simulink model "afe_inv_psm_with_hf_models"  (R2026a)
settings: Solver=ode23tb  StopTime=simlength  FixedStep=tc  MaxStep=glb_time.tc
values from neighbouring files (symbols this model uses):
  afe_ctrl = ctrl_afe_setup(glb_time.ts_afe, grid_emu.omega_grid_nom)    [init_model.m]
  afe_pwm_phase_shift_mod1 = 0    [init_model.m]
  CTRPIFF_CLIP_RELEASE = 0.001    [init_model.m]
  DThs_init = 0    [init_model.m]
  filters = setup_global_filters(glb_time.ts_afe, glb_time.ts_inv, glb_time.ts_dab, glb_time.tc)    [init_model.m]
  frt_data = frt_settings(test_index, test_subindex, asymmetric_error_type,      enable_frt_1, enable_frt_2, start_time_LVRT, deepPOSxi, deepPOSeta, deepNEGxi, deepNEGeta)    [init_model.m]
  glb_time = timing_setup(fpwm_afe, trgo_afe, fpwm_inv, trgo_inv, fpwm_single_phase_inv, trgo_single_phase_inv, fpwm_dab, trgo_dab,      fpwm_psfbc, trgo_psfbc, fpwm_isop_rail, trgo_isop_rail, fpwm_cllc, trgo_cllc, t_measure, tc_factor, tc_decimation, delay_pwm, dead_time_afe,      dead_time_inv, dead_time_single_phase_inv, dead_time_dab, dead_time_psfbc, dead_time_isop_rail, dead_time_cllc)    [init_model.m]
  grid_emu = grid_three_phase_emulator('Dyn11', delta_star, grid_nominal_power, application_voltage, us1, us2, fgrid,                  eq_grid_inductance, eq_grid_resistance, eta, ucc, i1m, p_iron, n1, n2, core_area, core_length, mur,                  up_xi_pu_ref, up_eta_pu_ref, un_xi_pu_ref, un_eta_pu_ref)    [init_model.m]
  i_react_pos_ref_2 = -ixi_ref_mod1*tan(acos(0.95))    [init_model.m]
  i_react_pos_ref_3 = ixi_ref_mod1*tan(acos(0.95))    [init_model.m]
  inv_pwm_phase_shift_mod1 = 0    [init_model.m]
  ixi_ref_mod1 = -0.85    [init_model.m]
  ki_align = 18    [init_model.m]
  kp_align = 0.25    [init_model.m]
  lim_down_align = -0.05    [init_model.m]
  lim_up_align = 0.05    [init_model.m]
  mavarage_filter_frequency_base_order = 2    [init_model.m]
  omega_m_sim = psm.omega_m_bez    [init_model.m]
  psm = psm_calculus_with_variants(application_voltage)    [init_model.m]
  psm_ctrl = ctrl_pmsm_setup(glb_time.ts_inv, psm.omega_bez, u_psm_scale, psm.Jm_norm)    [init_model.m]
  rms_tc = rms_filter_setup(rms_tc_obj)    [init_model.m]
  simlength = 1.75    [init_model.m]
  Tambient = 40    [init_model.m]
  time_aux_power_supply_fault = 1e3    (= 1000)    [init_model.m]
  time_gain_afe_module_1 = 1.0002    [init_model.m]
  time_gain_inv_module_2 = 1.001    [init_model.m]
  time_i_react_pos_ref_1 = start_time_LVRT + error_length + 0.335    [init_model.m]
  time_i_react_pos_ref_2 = time_i_react_pos_ref_1 + 0.5    (= 0.5)    [init_model.m]
  time_start_motor_control = 0.25    [init_model.m]
  torque_overload_factor = 1    [init_model.m]
  u_cm_comp_mod1 = 0    [init_model.m]
  u_psm_scale_ekf = sqrt(3)/2 * 2/3 * hwdata.inv.udc_nom/psm.ubez    [init_model.m]
undefined symbols (not defined in the file or in its folder): hf_power_cable_model, hwdata, magnitude, omega_m_bez, rpm_base, torque_base
libraries: fl_lib x136, nesl_utility x57, moving_average_filter x10, moving_average_filter_cc x8, ee_lib x5, sl_discontinuities x3, single_phase_transformer_lib x3, linear_double_integrator_observer_ccaller x2, discrete_time_low_pass_filter x2, threephase_inductor_lib x2, three_phase_pwm_modulator x2, three_phase_inverter_ideal_switch_based_model x2
(part 10 of 10)

== matlab function afe_inv_psm_with_hf_models/afe_abc_inv_psm_mod1/brake/MATLAB Function ==
  data: u input; y output; udc_ref input
function y = fcn(u,udc_ref)

persistent enable_brake

udc_brake_min = 1.15;
udc_brake_max = 1.175;

if isempty(enable_brake)
    enable_brake = 0
end

if u >= udc_ref*udc_brake_max
    y = 15;
    enable_brake = 1;
elseif (u < udc_ref*udc_brake_max && u >= udc_ref*udc_brake_min && enable_brake == 1)
    y = 15;
    enable_brake = 1;
elseif (u < udc_ref*udc_brake_max && u >= udc_ref*udc_brake_min && enable_brake == 0)
    y = 0;
    enable_brake = 0;
else
    y = 0;
    enable_brake = 0;
end

% function y = fcn(u,udc_ref)
% 
% persistent enable_brake
% 
% udc_brake_min = 1.145;
% udc_brake_max = 1.165;
% 
% if isempty(enable_brake)
%     enable_brake = 0
% end
% 
% if u >= udc_ref*udc_brake_max
%     y = 15;
%     enable_brake = 1;
% elseif (u < udc_ref*udc_brake_max && u >= udc_ref*udc_brake_min && enable_brake == 1)
%     y = 15;
%     enable_brake = 1;
% elseif (u < udc_ref*udc_brake_max && u >= udc_ref*udc_brake_min && enable_brake == 0)
%     y = 0;
%     enable_brake = 0;
% else
%     y = 0;
%     enable_brake = 0;
end

== matlab function afe_inv_psm_with_hf_models/afe_abc_inv_psm_mod1/AFE_control/afe_control/grid_voltage_phase_lock_loops/FHT-PLL/pll_stageB/double_integrator_observer/bounder1 ==
  data: u input; y output
function y = bounder(u)
    
    y = -pi + mod(u+3*pi,2*pi);
    
end

== matlab function afe_inv_psm_with_hf_models/afe_abc_inv_psm_mod1/AFE_control/afe_control/grid_voltage_phase_lock_loops/FHT-PLL/pll_stageB/double_integrator_observer/bounder2 ==
  data: u input; y output
function y = bounder(u)
    
    y = -pi + mod(u+3*pi,2*pi);
    
end

== matlab function afe_inv_psm_with_hf_models/afe_abc_inv_psm_mod1/INV_control/inverter_control/current_ctrl/bemf_observer/EKF_bemf_observer/extended_kalman_observer/double_integrator_observer/bounder2 ==
  data: u input; y output
function y = bounder(u)
    y = -pi + mod(u+3*pi,2*pi);
end

== matlab function afe_inv_psm_with_hf_models/afe_abc_inv_psm_mod1/AFE_control/afe_control/grid_voltage_phase_lock_loops/FHT-PLL_simulink/pll_stageA/filter_and_transformation/abc2alphabeta ==
  data: a input; alpha output; b input; c input; beta output
function [alpha,beta] = abc2alphabeta(a,b,c)

alpha = 2/3*(a - 1/2*b - 1/2*c);
beta  = 1/sqrt(3)*(b - c);

end

== matlab function afe_inv_psm_with_hf_models/afe_abc_inv_psm_mod1/AFE_control/afe_control/grid_voltage_phase_lock_loops/FHT-PLL_simulink/pll_stageA/sequences/alphabeta2xieta ==
  data: alpha input; xi output; beta input; gamma input; eta output
function [xi,eta] = alphabeta2xieta_pos(alpha,beta,gamma)

    xi  =  (alpha*cos(gamma) + beta*sin(gamma));
    eta = (-alpha*sin(gamma) + beta*cos(gamma));

end

== matlab function afe_inv_psm_with_hf_models/afe_abc_inv_psm_mod1/AFE_control/afe_control/grid_voltage_phase_lock_loops/FHT-PLL_simulink/pll_stageB/bounder1 ==
  data: u input; y output
function y = bounder(u)
    y = -pi + mod(u+3*pi,2*pi);
end

== matlab function afe_inv_psm_with_hf_models/afe_abc_inv_psm_mod1/AFE_control/afe_control/grid_voltage_phase_lock_loops/FHT-PLL_simulink/pll_stageB/double_integrator_observer/bounder1 ==
  data: u input; y output
function y = bounder(u)
    
    y = -pi + mod(u+3*pi,2*pi);
    
end

== matlab function afe_inv_psm_with_hf_models/afe_abc_inv_psm_mod1/AFE_control/afe_control/grid_voltage_phase_lock_loops/dq_pll/pll_stageA/mormalization_and_transformation/abc2alphabeta ==
  data: a input; alpha output; b input; c input; beta output
function [alpha,beta] = abc2alphabeta(a,b,c)

alpha = 2/3*(a - 1/2*b - 1/2*c);
beta  = 1/sqrt(3)*(b - c);

end

== matlab function afe_inv_psm_with_hf_models/afe_abc_inv_psm_mod1/AFE_control/afe_control/grid_voltage_phase_lock_loops/dq_pll/pll_stageA/sequences/alphabeta2xieta/alphabeta2xieta_neg ==
  data: alpha input; xi output; beta input; gamma input; eta output
function [xi,eta] = alphabeta2xieta_neg(alpha,beta,gamma)

    xi  = alpha*cos(gamma) - beta*sin(gamma);
    eta = alpha*sin(gamma) + beta*cos(gamma);

end

== matlab function afe_inv_psm_with_hf_models/afe_abc_inv_psm_mod1/AFE_control/afe_control/grid_voltage_phase_lock_loops/dq_pll/pll_stageA/sequences/alphabeta2xieta/alphabeta2xieta_pos ==
  data: alpha input; xi output; beta input; gamma input; eta output
function [xi,eta] = alphabeta2xieta_pos(alpha,beta,gamma)

    xi  =  alpha*cos(gamma) + beta*sin(gamma);
    eta = -alpha*sin(gamma) + beta*cos(gamma);

end

== matlab function afe_inv_psm_with_hf_models/afe_abc_inv_psm_mod1/INV_control/inverter_control/current_ctrl/bemf_observer/bemf_observer/double_integrator_observer/bounder1 ==
  data: u input; y output
function y = bounder(u)
    
    y = -pi + mod(u+3*pi,2*pi);
end

== matlab function afe_inv_psm_with_hf_models/afe_abc_inv_psm_mod1/INV_control/inverter_control/current_ctrl/bemf_observer/bemf_observer/double_integrator_observer/bounder2 ==
  data: u input; y output
function y = bounder(u)
    
    u = -pi + mod(u+3*pi,2*pi);
    
    y = u;
end

== matlab function afe_inv_psm_with_hf_models/afe_abc_inv_psm_mod1/AFE_control/afe_control/FRT-VDE4110/FRT-PosNegReactiveCurrentReferences/avg_flt_500ms/avg_flt_1 ==
  data: x input; y1 output; w input; ts input; enable input
function y1  = avg_flt(x,w,ts, enable)

    persistent x_int x_int_1 y_N N

    N = (1/(w/(2*pi)))/ts+1;

    if isempty(x_int)
        x_int_1 = 0;
        y_N = zeros(1,N);
        y1 = 0;
    end


    if enable == 1
        x_int = x * ts * w + x_int_1;
        x_int_1 = x_int;
        y_N(1,1) = x_int;
        y1 = 1/(2*pi)*((y_N(1,1) - y_N(1,N)));
        for i = 1:(N-1)
            y_N(1,N+1-i) = y_N(1,N-i); 
        end
    else
        y1 = 1/(2*pi)*((y_N(1,1) - y_N(1,N)));
    end
end

== matlab function afe_inv_psm_with_hf_models/afe_abc_inv_psm_mod1/AFE_control/afe_control/grid_voltage_phase_lock_loops/dq_pll/pll_stageB/double_integrator_observer/bounder1 ==
  data: u input; y output
function y = bounder(u)
    
    y = -pi + mod(u+3*pi,2*pi);
    
end

== matlab function afe_inv_psm_with_hf_models/afe_abc_inv_psm_mod1/AFE_control/afe_control/islanding_mode_detector/MATLAB Function ==
  data: alpha input; xi output; beta input; gamma input; eta output
function [xi,eta] = alphabeta2pos(alpha,beta,gamma)

    xi  =  alpha*cos(gamma) + beta*sin(gamma);
    eta = -alpha*sin(gamma) + beta*cos(gamma);

end

== matlab function afe_inv_psm_with_hf_models/afe_abc_inv_psm_mod1/AFE_control/afe_control/grid_voltage_phase_lock_loops/dq_pll/pll_stageB/double_integrator_observer/bounder2 ==
  data: u input; y output
function y = bounder(u)
    
    y = -pi + mod(u+3*pi,2*pi);
    
end

== matlab function afe_inv_psm_with_hf_models/afe_abc_inv_psm_mod1/AFE_control/afe_control/islanding_mode_detector/bounder ==
  data: u input; y output
function y = bounder(u)
    
    u = -pi + mod(u+3*pi,2*pi);
    
    y = u;
end

== matlab function afe_inv_psm_with_hf_models/afe_abc_inv_psm_mod1/AFE_control/afe_control/current_ctrl/inner_current_ctrl/zero_current_ctrl/antiwind_up/MATLAB Function1 ==
  data: da input; das output; db input; dc input; scaling input; dbs output; dcs output
function [das, dbs, dcs] = fcn(da,db,dc,scaling)

das = da/scaling;
dbs = db/scaling;
dcs = dc/scaling;

== matlab function afe_inv_psm_with_hf_models/afe_abc_inv_psm_mod1/AFE_control/afe_control/FRT-VDE4110/FRT-PosNegReactiveCurrentReferences/avg_flt_500ms1/avg_flt_1 ==
  data: x input; y1 output; w input; ts input; enable input
function y1  = avg_flt(x,w,ts, enable)

    persistent x_int x_int_1 y_N N

    N = (1/(w/(2*pi)))/ts+1;

    if isempty(x_int)
        x_int_1 = 0;
        y_N = zeros(1,N);
        y1 = 0;
    end


    if enable == 1
        x_int = x * ts * w + x_int_1;
        x_int_1 = x_int;
        y_N(1,1) = x_int;
        y1 = 1/(2*pi)*((y_N(1,1) - y_N(1,N)));
        for i = 1:(N-1)
            y_N(1,N+1-i) = y_N(1,N-i); 
        end
    else
        y1 = 1/(2*pi)*((y_N(1,1) - y_N(1,N)));
    end
end

== matlab function afe_inv_psm_with_hf_models/afe_abc_inv_psm_mod1/AFE_control/afe_control/FRT-VDE4110/FRT-PosNegReactiveCurrentReferences/avg_flt_500ms2/avg_flt_1 ==
  data: x input; y1 output; w input; ts input; enable input
function y1  = avg_flt(x,w,ts, enable)

    persistent x_int x_int_1 y_N N

    N = (1/(w/(2*pi)))/ts+1;

    if isempty(x_int)
        x_int_1 = 0;
        y_N = zeros(1,N);
        y1 = 0;
    end


    if enable == 1
        x_int = x * ts * w + x_int_1;
        x_int_1 = x_int;
        y_N(1,1) = x_int;
        y1 = 1/(2*pi)*((y_N(1,1) - y_N(1,N)));
        for i = 1:(N-1)
            y_N(1,N+1-i) = y_N(1,N-i); 
        end
    else
        y1 = 1/(2*pi)*((y_N(1,1) - y_N(1,N)));
    end
end

== matlab function afe_inv_psm_with_hf_models/afe_abc_inv_psm_mod1/AFE_control/afe_control/FRT-VDE4110/FRT-PosNegReactiveCurrentReferences/avg_flt_500ms3/avg_flt_1 ==
  data: x input; y1 output; w input; ts input; enable input
function y1  = avg_flt(x,w,ts, enable)

    persistent x_int x_int_1 y_N N

    N = (1/(w/(2*pi)))/ts+1;

    if isempty(x_int)
        x_int_1 = 0;
        y_N = zeros(1,N);
        y1 = 0;
    end


    if enable == 1
        x_int = x * ts * w + x_int_1;
        x_int_1 = x_int;
        y_N(1,1) = x_int;
        y1 = 1/(2*pi)*((y_N(1,1) - y_N(1,N)));
        for i = 1:(N-1)
            y_N(1,N+1-i) = y_N(1,N-i); 
        end
    else
        y1 = 1/(2*pi)*((y_N(1,1) - y_N(1,N)));
    end
end

== matlab function afe_inv_psm_with_hf_models/afe_abc_inv_psm_mod1/AFE_control/afe_control/grid_voltage_sequences/v_alphabeta2xieta/MATLAB Function ==
  data: alpha input; xi output; beta input; gamma input; eta output
function [xi,eta] = alphabeta2pos(alpha,beta,gamma)

    xi  =  alpha*cos(gamma) + beta*sin(gamma);
    eta = -alpha*sin(gamma) + beta*cos(gamma);

end

== matlab function afe_inv_psm_with_hf_models/afe_abc_inv_psm_mod1/AFE_control/afe_control/grid_voltage_sequences/v_alphabeta2xieta/MATLAB Function1 ==
  data: alpha input; xi output; beta input; gamma input; eta output
function [xi,eta] = alphabeta2neg(alpha,beta,gamma)

    xi  = alpha*cos(gamma) - beta*sin(gamma);
    eta = alpha*sin(gamma) + beta*cos(gamma);

end

== matlab function afe_inv_psm_with_hf_models/afe_abc_inv_psm_mod1/AFE_control/afe_control/grid_voltage_sequences/grid_voltage_sampling_and_alpha_beta_transformation/v_abc2alphabeta ==
  data: v_abc input; alpha output; beta output
function [alpha,beta] = abc2alphabeta(v_abc)

alpha = 2/3*(v_abc(1) - 1/2*v_abc(2) - 1/2*v_abc(3));
beta  = 1/sqrt(3)*(v_abc(2) - v_abc(3));

end

== matlab function afe_inv_psm_with_hf_models/afe_abc_inv_psm_mod1/AFE_control/afe_control/grid_current_sequences_and_reactive_pwr_ctrl/i_alphabeta2xieta/MATLAB Function ==
  data: alpha input; xi output; beta input; gamma input; eta output
function [xi,eta] = alphabeta2pos(alpha,beta,gamma)

    xi  =  alpha*cos(gamma) + beta*sin(gamma);
    eta = -alpha*sin(gamma) + beta*cos(gamma);

end

== matlab function afe_inv_psm_with_hf_models/afe_abc_inv_psm_mod1/AFE_control/afe_control/grid_current_sequences_and_reactive_pwr_ctrl/i_alphabeta2xieta/MATLAB Function1 ==
  data: alpha input; xi output; beta input; gamma input; eta output
function [xi,eta] = alphabeta2neg(alpha,beta,gamma)

    xi  = alpha*cos(gamma) - beta*sin(gamma);
    eta = alpha*sin(gamma) + beta*cos(gamma);

end

== matlab function afe_inv_psm_with_hf_models/afe_abc_inv_psm_mod1/AFE_control/afe_control/grid_current_sequences_and_reactive_pwr_ctrl/grid_current_sampling_and_alpha_beta_transformation/i_abc2alphabeta ==
  data: i_abc input; alpha output; beta output
function [alpha,beta] = abc2alphabeta(i_abc)

alpha = 2/3*(i_abc(1) - 1/2*i_abc(2) - 1/2*i_abc(3));
beta  = 1/sqrt(3)*(i_abc(2) - i_abc(3));

end

== matlab function afe_inv_psm_with_hf_models/afe_abc_inv_psm_mod1/AFE_control/afe_control/current_ctrl/xieta2abc/MATLAB Function2 ==
  data: alpha input; a output; beta input; b output; c output
function [a,b,c] = alphabeta2abc(alpha,beta)

a = alpha;
b = -(1/2)*alpha + sqrt(3)/2*beta;
c = -(1/2)*alpha - sqrt(3)/2*beta;

end

== matlab function afe_inv_psm_with_hf_models/afe_abc_inv_psm_mod1/AFE_control/afe_control/current_ctrl/xieta2abc/Negative Sequence ==
  data: xi input; alpha output; eta input; phase input; beta output
function [alpha,beta] = neg2alphabeta(xi,eta,phase)

    alpha = xi*cos(phase)  + eta*sin(phase);
    beta  = -xi*sin(phase) + eta*cos(phase);

end

== matlab function afe_inv_psm_with_hf_models/afe_abc_inv_psm_mod1/AFE_control/afe_control/current_ctrl/xieta2abc/Positive Sequence ==
  data: xi input; alpha output; eta input; phase input; beta output
function [alpha,beta] = pos2alphabeta(xi,eta,phase)

    alpha = xi*cos(phase) - eta*sin(phase);
    beta  = xi*sin(phase) + eta*cos(phase);

end

== matlab function afe_inv_psm_with_hf_models/afe_abc_inv_psm_mod1/AFE_control/afe_control/grid_voltage_phase_lock_loops/dq_pll/pll_stageB/bounder1 ==
  data: u input; y output
function y = bounder(u)
    y = -pi + mod(u+3*pi,2*pi);
end

== matlab function afe_inv_psm_with_hf_models/afe_abc_inv_psm_mod1/INV_control/inverter_control/encoder-sensorless-switch/MATLAB Function ==
  data: omega_ctrl output; phase_psm input; omega_obs input; phase_obs input; phase_ctrl output; omega_psm input; omega_th input
function [omega_ctrl, phase_ctrl] = switch_enc2obs(phase_psm, omega_obs, phase_obs, omega_psm, omega_th)

if abs(omega_psm) > omega_th
    omega_ctrl = omega_obs;
    phase_ctrl = phase_obs;
else
    omega_ctrl = omega_psm;
    phase_ctrl = phase_psm;
end

== matlab function afe_inv_psm_with_hf_models/afe_abc_inv_psm_mod1/INV_control/inverter_control/current_ctrl/bemf_observer/EKF_bemf_observer/extended_kalman_observer/double_integrator_observer/bounder1 ==
  data: u input; y output
function y = bounder(u)
    y = -pi + mod(u+3*pi,2*pi);
end

== matlab function afe_inv_psm_with_hf_models/afe_abc_inv_psm_mod1/AFE_control/afe_control/grid_voltage_phase_lock_loops/FHT-PLL_simulink/pll_stageB/double_integrator_observer/bounder2 ==
  data: u input; y output
function y = bounder(u)
    
    y = -pi + mod(u+3*pi,2*pi);
    
end

== matlab function afe_inv_psm_with_hf_models/afe_abc_inv_psm_mod1/INV_control/inverter_control/encoder-sensorless-switch/double_integrator_observer/bounder1 ==
  data: u input; y output
function y = bounder(u)
    y = -pi + mod(u+3*pi,2*pi);
end

== matlab function afe_inv_psm_with_hf_models/afe_abc_inv_psm_mod1/INV_control/inverter_control/encoder-sensorless-switch/double_integrator_observer/bounder2 ==
  data: u input; y output
function y = bounder(u)
    y = -pi + mod(u+3*pi,2*pi);
end

== matlab function afe_inv_psm_with_hf_models/afe_abc_inv_psm_mod1/AFE_control/afe_control/current_ctrl/inner_current_ctrl/zero_current_ctrl/antiwind_up/MATLAB Function2 ==
  data: a input; alpha output; b input; c input; beta output; gamma output
function [alpha,beta, gamma] = abc2alphabeta(a,b,c)

alpha = 2/3*(a - 1/2*b - 1/2*c);
beta  = 1/sqrt(3)*(b - c);
gamma = (a+b+c)/3;

end

== matlab function afe_inv_psm_with_hf_models/afe_abc_inv_psm_mod1/AFE_control/afe_control/grid_voltage_phase_lock_loops/FHT-PLL/pll_stageA/filter_and_transformation/abc2alphabeta ==
  data: a input; alpha output; b input; c input; beta output
function [alpha,beta] = abc2alphabeta(a,b,c)

alpha = 2/3*(a - 1/2*b - 1/2*c);
beta  = 1/sqrt(3)*(b - c);

end

== matlab function afe_inv_psm_with_hf_models/afe_abc_inv_psm_mod1/AFE_control/afe_control/grid_voltage_phase_lock_loops/FHT-PLL/pll_stageA/sequences/alphabeta2xieta ==
  data: alpha input; xi output; beta input; gamma input; eta output
function [xi,eta] = alphabeta2xieta_pos(alpha,beta,gamma)

    xi  =  (alpha*cos(gamma) + beta*sin(gamma));
    eta = (-alpha*sin(gamma) + beta*cos(gamma));

end

== matlab function afe_inv_psm_with_hf_models/afe_abc_inv_psm_mod1/INV_control/inverter_control/current_ctrl/current_transformation/alphabeta2dq ==
  data: alpha input; d output; beta input; gamma input; q output
function [d,q] = alphabeta2dq(alpha,beta,gamma)

    d  =  alpha*cos(gamma) + beta*sin(gamma);
    q = -alpha*sin(gamma) + beta*cos(gamma);

end

== matlab function afe_inv_psm_with_hf_models/afe_abc_inv_psm_mod1/AFE_control/afe_control/current_ctrl/current_transformation/uvw2alphabeta ==
  data: u input; alpha output; v input; w input; beta output
function [alpha,beta] = uvw2alphabeta(u,v,w)

alpha = 2/3*(u - 1/2*v - 1/2*w);
beta  = 2/3*(sqrt(3)/2*(v - w));

end
